simulink model "sens_acq_gnss"  (R2026b)
settings: Solver=VariableStepAuto
values from neighbouring files (symbols this model uses):
  D = zeros(nx, ny, 'uint8')    [sens_lidar2d_fast.m]
  P = (P + P.')/2    [sens_nav_ekf.m]
libraries: ros2lib x3, simulink x2, robotcorelib x1
settings Model: Creator=aomar  LastModifiedBy=aomar

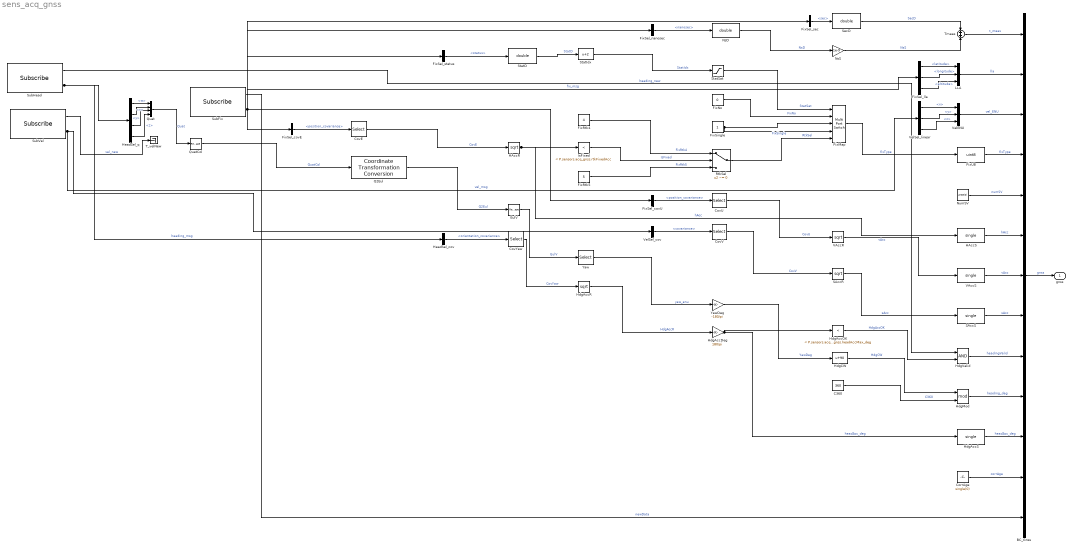
== system sens_acq_gnss ==
  BC_Gnss : BusCreator  Inputs=13  OutDataTypeStr=Bus: Bus_GnssRaw  NonVirtualBus=on
      settings: InheritFromInputs=off
  C360 : Constant  Value=360
  CorrAge : Constant  Value=single(0)  OutDataTypeStr=single
  CovE : Selector  InputPortWidth=9  IndexOptions=Index vector (dialog)  Indices=1  OutputSizes=1
  CovU : Selector  InputPortWidth=9  IndexOptions=Index vector (dialog)  Indices=9  OutputSizes=1
  CovV : Selector  InputPortWidth=36  IndexOptions=Index vector (dialog)  Indices=1  OutputSizes=1
  CovYaw : Selector  InputPortWidth=9  IndexOptions=Index vector (dialog)  Indices=9  OutputSizes=1
  EulV : Reshape
  FixMap : MultiPortSwitch  Inputs=4  SaturateOnIntegerOverflow=off  InputSameDT=off
  FixNo : Constant  Value=0
  FixRtk4 : Constant  Value=4
  FixRtk5 : Constant  Value=5
  FixSel_covE : BusSelector  OutputSignals=position_covariance
  FixSel_covU : BusSelector  OutputSignals=position_covariance
  FixSel_lla : BusSelector  OutputSignals=latitude,longitude,altitude
  FixSel_nanosec : BusSelector  OutputSignals=header.stamp.nanosec
  FixSel_sec : BusSelector  OutputSignals=header.stamp.sec
  FixSel_status : BusSelector  OutputSignals=status.status
  FixSingle : Constant
  FixU8 : DataTypeConversion  OutDataTypeStr=uint8  RndMeth=Floor
  HAccR : Math  Operator=sqrt
  HAccS : DataTypeConversion  OutDataTypeStr=single  RndMeth=Floor
  HdgAccDeg : Gain  Gain=180/pi
  HdgAccOK : simulink/Logic and Bit Operations/Compare To Constant  relop=<  const=P.sensors.acq_gnss.headAccMax_deg  OutDataTypeStr=boolean
  HdgAccR : Math  Operator=sqrt
  HdgAccS : DataTypeConversion  OutDataTypeStr=single  RndMeth=Floor
  HdgCW : Bias  Bias=90  SaturateOnIntegerOverflow=off
  HdgMod : Math  Operator=mod
  HdgValid : Logic  AllPortsSameDT=off  OutDataTypeStr=boolean
  HeadSel_cov : BusSelector  OutputSignals=orientation_covariance
  HeadSel_q : BusSelector  OutputSignals=orientation.w,orientation.x,orientation.y,orientation.z
  IsFixed : simulink/Logic and Bit Operations/Compare To Constant  relop=<  const=P.sensors.acq_gnss.rtkFixedAcc  OutDataTypeStr=boolean
  LLA : Concatenate  NumInputs=3
  NsD : DataTypeConversion  OutDataTypeStr=double  RndMeth=Floor
  NsS : Gain  Gain=1e-9
  NumSV : Constant  Value=uint8(0)  OutDataTypeStr=uint8
  Q2Eul : robotcorelib/Coordinate Transformation Conversion  InputRepresentation=Quaternion  InputEulerSequence=ZYX  ShowTrVecInputPort=on  OutputRepresentation=Euler Angles  OutputEulerSequence=ZYX  ShowTrVecOutputPort=on  SimulateUsing=Interpreted execution
      settings: LibrarySourceBlock=navlib/Utilities/Coordinate Transformation Conversion
  Quat : Concatenate  NumInputs=4
  QuatCol : Reshape  OutputDimensionality=Column vector (2-D)
  RtkSel : Switch  Criteria=u2 ~= 0  SaturateOnIntegerOverflow=off  InputSameDT=off
  SAccR : Math  Operator=sqrt
  SAccS : DataTypeConversion  OutDataTypeStr=single  RndMeth=Floor
  SecD : DataTypeConversion  OutDataTypeStr=double  RndMeth=Floor
  StatD : DataTypeConversion  OutDataTypeStr=double  RndMeth=Floor
  StatIdx : Bias  Bias=2  SaturateOnIntegerOverflow=off
  StatSat : Saturate  UpperLimit=4  LowerLimit=1
  SubFix : ros2lib/Subscribe  topicSource=Specify your own  topic=/fix  messageType=sensor_msgs/NavSatFix  SubscriberMode=At sample time  sampleTime=P.sensors.acq_gnss.Ts  CallbackGroupType=Default  CallbackGroupName=callback_group_1  QOSHistory=Keep last  QOSDepth=10  QOSReliability=Reliable  QOSDurability=Volatile  QOSDeadline=Inf  QOSLifespan=Inf  QOSLiveliness=Automatic  QOSLeaseDuration=Inf  QOSAvoidROSNamespaceConventions=off
  SubHead : ros2lib/Subscribe  topicSource=Specify your own  topic=/navheading  messageType=sensor_msgs/Imu  SubscriberMode=At sample time  sampleTime=P.sensors.acq_gnss.Ts  CallbackGroupType=Default  CallbackGroupName=callback_group_1  QOSHistory=Keep last  QOSDepth=10  QOSReliability=Reliable  QOSDurability=Volatile  QOSDeadline=Inf  QOSLifespan=Inf  QOSLiveliness=Automatic  QOSLeaseDuration=Inf  QOSAvoidROSNamespaceConventions=off
  SubVel : ros2lib/Subscribe  topicSource=Specify your own  topic=/fix_velocity  messageType=geometry_msgs/TwistWithCovarianceStamped  SubscriberMode=At sample time  sampleTime=P.sensors.acq_gnss.Ts  CallbackGroupType=Default  CallbackGroupName=callback_group_1  QOSHistory=Keep last  QOSDepth=10  QOSReliability=Reliable  QOSDurability=Volatile  QOSDeadline=Inf  QOSLifespan=Inf  QOSLiveliness=Automatic  QOSLeaseDuration=Inf  QOSAvoidROSNamespaceConventions=off
  T_velNew : Terminator
  Tmeas : Sum
  VAccR : Math  Operator=sqrt
  VAccS : DataTypeConversion  OutDataTypeStr=single  RndMeth=Floor
  VelENU : Concatenate  NumInputs=3
  VelSel_cov : BusSelector  OutputSignals=twist.covariance
  VelSel_linear : BusSelector  OutputSignals=twist.twist.linear.x,twist.twist.linear.y,twist.twist.linear.z
  Yaw : Selector  InputPortWidth=3  IndexOptions=Index vector (dialog)  Indices=1  OutputSizes=1
  YawDeg : Gain  Gain=-180/pi
  gnss : Outport  OutDataTypeStr=Bus: Bus_GnssRaw
  wires:
  SubHead/1 -> HdgValid/1  "heading_new"
  SubHead/2 -> HeadSel_cov/1, HeadSel_q/1  "heading_msg"
  SubVel/1 -> T_velNew/1  "vel_new"
  SubVel/2 -> VelSel_cov/1, VelSel_linear/1  "vel_msg"
  HeadSel_q/1 -> Quat/1  "<w>"
  HeadSel_q/2 -> Quat/2  "<x>"
  HeadSel_q/3 -> Quat/3  "<y>"
  HeadSel_q/4 -> Quat/4  "<z>"
  Quat/1 -> QuatCol/1  "Quat"
  QuatCol/1 -> Q2Eul/1  "QuatCol"
  SubFix/1 -> BC_Gnss/13  "newData"
  SubFix/2 -> FixSel_covU/1, FixSel_sec/1, FixSel_nanosec/1, FixSel_status/1, FixSel_lla/1, FixSel_covE/1  "fix_msg"
  FixSel_covE/1 -> CovE/1  "<position_covariance>"
  CovE/1 -> HAccR/1  "CovE"
  Q2Eul/1 -> EulV/1  "Q2Eul"
  FixSel_status/1 -> StatD/1  "<status>"
  HeadSel_cov/1 -> CovYaw/1  "<orientation_covariance>"
  HAccR/1 -> HAccS/1, IsFixed/1  "hAcc"
  EulV/1 -> Yaw/1  "EulV"
  CovYaw/1 -> HdgAccR/1  "CovYaw"
  StatD/1 -> StatIdx/1  "StatD"
  FixRtk4/1 -> RtkSel/1  "FixRtk4"
  IsFixed/1 -> RtkSel/2  "IsFixed"
  FixRtk5/1 -> RtkSel/3  "FixRtk5"
  HdgAccR/1 -> HdgAccDeg/1  "HdgAccR"
  StatIdx/1 -> StatSat/1  "StatIdx"
  Yaw/1 -> YawDeg/1  "yaw_enu"
  FixSel_nanosec/1 -> NsD/1  "<nanosec>"
  FixSel_covU/1 -> CovU/1  "<position_covariance>"
  VelSel_cov/1 -> CovV/1  "<covariance>"
  StatSat/1 -> FixMap/1  "StatSat"
  FixNo/1 -> FixMap/2  "FixNo"
  FixSingle/1 -> FixMap/3, FixMap/4  "FixSingle"
  YawDeg/1 -> HdgCW/1  "YawDeg"
  HdgAccDeg/1 -> HdgAccS/1, HdgAccOK/1  "headAcc_deg"
  CovU/1 -> VAccR/1  "CovU"
  CovV/1 -> SAccR/1  "CovV"
  RtkSel/1 -> FixMap/5  "RtkSel"
  NsD/1 -> NsS/1  "NsD"
  FixSel_sec/1 -> SecD/1  "<sec>"
  NsS/1 -> Tmeas/2  "NsS"
  VAccR/1 -> VAccS/1  "vAcc"
  SAccR/1 -> SAccS/1  "sAcc"
  HdgAccOK/1 -> HdgValid/2  "HdgAccOK"
  C360/1 -> HdgMod/2  "C360"
  FixMap/1 -> FixU8/1  "fixType"
  HdgCW/1 -> HdgMod/1  "HdgCW"
  SecD/1 -> Tmeas/1  "SecD"
  FixSel_lla/1 -> LLA/1  "<latitude>"
  FixSel_lla/2 -> LLA/2  "<longitude>"
  FixSel_lla/3 -> LLA/3  "<altitude>"
  VelSel_linear/1 -> VelENU/1  "<x>"
  VelSel_linear/2 -> VelENU/2  "<y>"
  VelSel_linear/3 -> VelENU/3  "<z>"
  LLA/1 -> BC_Gnss/2  "lla"
  VelENU/1 -> BC_Gnss/3  "vel_ENU"
  Tmeas/1 -> BC_Gnss/1  "t_meas"
  NumSV/1 -> BC_Gnss/5  "numSV"
  HdgValid/1 -> BC_Gnss/9  "headingValid"
  HdgMod/1 -> BC_Gnss/10  "heading_deg"
  CorrAge/1 -> BC_Gnss/12  "corrAge"
  FixU8/1 -> BC_Gnss/4  "fixType"
  HAccS/1 -> BC_Gnss/6  "hAcc"
  VAccS/1 -> BC_Gnss/7  "vAcc"
  SAccS/1 -> BC_Gnss/8  "sAcc"
  HdgAccS/1 -> BC_Gnss/11  "headAcc_deg"
  BC_Gnss/1 -> gnss/1  "gnss"
